simulink model "snap_adc5g_spec_rpi"  (R2019a)
settings: Solver=VariableStepDiscrete  StartTime=0.0  StopTime=10.0  RelTol=1e-3
undefined symbols (not defined in the file): pfb_coeff_gen_calc
libraries: xbsIndex_r4 x13965, casper_library_misc x80, casper_library_delays x43, xps_library x5, xbsReplacements_r4 x2, casper_library_communications x1
(part 2 of 152)

== system snap_adc5g_spec_rpi/fft_shift ==
  sim_1 : Inport
  convert1_1 : DataTypeConversion  OutDataTypeStr=fixdt('ufix32_En0')  LockScale=on
  convert2_1 : DataTypeConversion  OutDataTypeStr=fixdt('ufix32_En0')  ConvertRealWorld=Stored Integer (SI)  LockScale=on
  gain_1 : Gain
  io_delay : xbsIndex_r4/Delay  rst=off  infoeditControl=Selection of Reset will increase slice count due to use of real FFs and instead of SRLs  en=off  latency=0  reg_retiming=on  dbl_ovrd=off  block_type=delay
  reint1 : xbsIndex_r4/Reinterpret  force_arith_type=on  arith_type=Unsigned  force_bin_pt=on  bin_pt=0  block_type=reinterpret
  slice_reg : xbsIndex_r4/Slice  nbits=32  boolean_output=off  mode=Lower Bit Location + Width  bit1=0  base1=MSB of Input  bit0=0  base0=LSB of Input  dbl_ovrd=off  block_type=slice
  snap_adc5g_spec_rpi_fft_shift_user_data_out : xbsIndex_r4/Gateway In  gui_display_data_type=Fixed-point  arith_type=Unsigned  n_bits=32  bin_pt=0  preci_type=Single  exp_width=8  frac_width=24  rows=1  columns=1  quantization="Round  (unbiased: +/- Inf)"  overflow=Saturate  period=1  UseAsADC=off  ADCChannel='1'  interface=None  automatic_assignment=on  address_offset=hex2dec('00')  intf_name=''  intf_description=''  default_value=0  timing_constraint=None  locs_specified=off  LOCs={}  io_standard={}  inherit_from_input=off  hdl_port=on  dbl_ovrd=off  block_type=gatewayin
  in_reg : Outport
  wires:
  snap_adc5g_spec_rpi_fft_shift_user_data_out/1 -> io_delay/1
  sim_1/1 -> convert1_1/1
  convert1_1/1 -> convert2_1/1
  convert2_1/1 -> gain_1/1
  gain_1/1 -> snap_adc5g_spec_rpi_fft_shift_user_data_out/1
  io_delay/1 -> slice_reg/1
  slice_reg/1 -> reint1/1
  reint1/1 -> in_reg/1

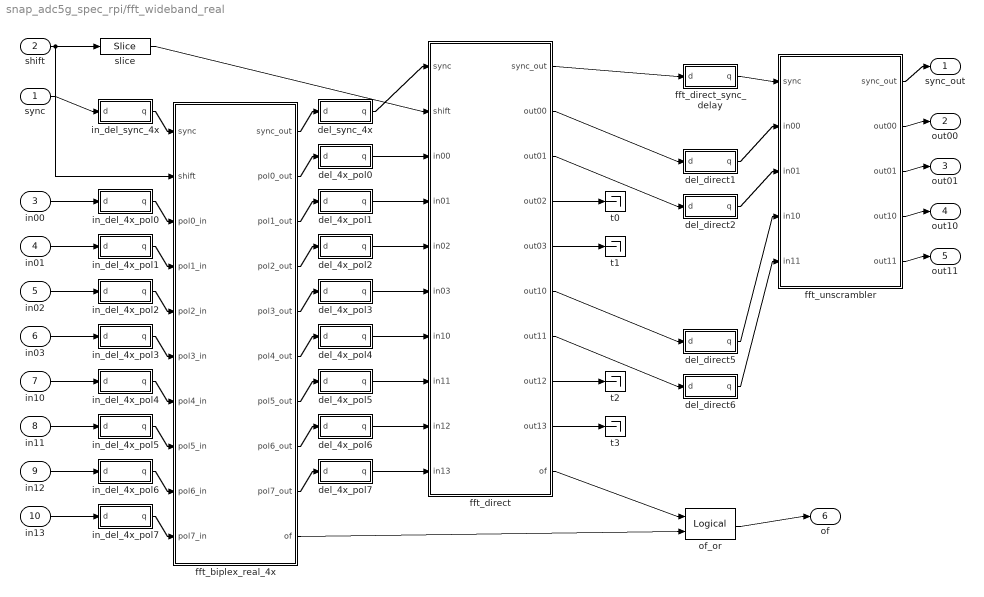
== system snap_adc5g_spec_rpi/fft_wideband_real ==
  sync : Inport
  shift : Inport  Port=2
  in00 : Inport  Port=3
  in01 : Inport  Port=4
  in02 : Inport  Port=5
  in03 : Inport  Port=6
  in10 : Inport  Port=7
  in11 : Inport  Port=8
  in12 : Inport  Port=9
  in13 : Inport  Port=10
  del_4x_pol0 : Subsystem  AncestorBlock=casper_library_delays/pipeline  mask(pipeline){csp_latency=0}
      mask prompts: csp_latency "Latency"
      mask help:
      | An explicitly laid-out delay line to avoid mapping to SRL16s
      | for use in pipelining to help achieve timing closure.
      mask init:
      | pipeline_init(gcb,'latency',csp_latency);
      settings: AttributesFormatString=Latency = %<latency>
      mask Display:
      | port_label('input', 1, 'd');
      | port_label('output', 1, 'q');
      | disp(['Z^-', num2str(csp_latency)]);
  del_4x_pol1 : Subsystem  AncestorBlock=casper_library_delays/pipeline  mask(pipeline){csp_latency=0}
      mask prompts: csp_latency "Latency"
      mask help:
      | An explicitly laid-out delay line to avoid mapping to SRL16s
      | for use in pipelining to help achieve timing closure.
      mask init:
      | pipeline_init(gcb,'latency',csp_latency);
      settings: AttributesFormatString=Latency = %<latency>
      mask Display:
      | port_label('input', 1, 'd');
      | port_label('output', 1, 'q');
      | disp(['Z^-', num2str(csp_latency)]);
  del_4x_pol2 : Subsystem  AncestorBlock=casper_library_delays/pipeline  mask(pipeline){csp_latency=0}
      mask prompts: csp_latency "Latency"
      mask help:
      | An explicitly laid-out delay line to avoid mapping to SRL16s
      | for use in pipelining to help achieve timing closure.
      mask init:
      | pipeline_init(gcb,'latency',csp_latency);
      settings: AttributesFormatString=Latency = %<latency>
      mask Display:
      | port_label('input', 1, 'd');
      | port_label('output', 1, 'q');
      | disp(['Z^-', num2str(csp_latency)]);
  del_4x_pol3 : Subsystem  AncestorBlock=casper_library_delays/pipeline  mask(pipeline){csp_latency=0}
      mask prompts: csp_latency "Latency"
      mask help:
      | An explicitly laid-out delay line to avoid mapping to SRL16s
      | for use in pipelining to help achieve timing closure.
      mask init:
      | pipeline_init(gcb,'latency',csp_latency);
      settings: AttributesFormatString=Latency = %<latency>
      mask Display:
      | port_label('input', 1, 'd');
      | port_label('output', 1, 'q');
      | disp(['Z^-', num2str(csp_latency)]);
  del_4x_pol4 : Subsystem  AncestorBlock=casper_library_delays/pipeline  mask(pipeline){csp_latency=0}
      mask prompts: csp_latency "Latency"
      mask help:
      | An explicitly laid-out delay line to avoid mapping to SRL16s
      | for use in pipelining to help achieve timing closure.
      mask init:
      | pipeline_init(gcb,'latency',csp_latency);
      settings: AttributesFormatString=Latency = %<latency>
      mask Display:
      | port_label('input', 1, 'd');
      | port_label('output', 1, 'q');
      | disp(['Z^-', num2str(csp_latency)]);
  del_4x_pol5 : Subsystem  AncestorBlock=casper_library_delays/pipeline  mask(pipeline){csp_latency=0}
      mask prompts: csp_latency "Latency"
      mask help:
      | An explicitly laid-out delay line to avoid mapping to SRL16s
      | for use in pipelining to help achieve timing closure.
      mask init:
      | pipeline_init(gcb,'latency',csp_latency);
      settings: AttributesFormatString=Latency = %<latency>
      mask Display:
      | port_label('input', 1, 'd');
      | port_label('output', 1, 'q');
      | disp(['Z^-', num2str(csp_latency)]);
  del_4x_pol6 : Subsystem  AncestorBlock=casper_library_delays/pipeline  mask(pipeline){csp_latency=0}
      mask prompts: csp_latency "Latency"
      mask help:
      | An explicitly laid-out delay line to avoid mapping to SRL16s
      | for use in pipelining to help achieve timing closure.
      mask init:
      | pipeline_init(gcb,'latency',csp_latency);
      settings: AttributesFormatString=Latency = %<latency>
      mask Display:
      | port_label('input', 1, 'd');
      | port_label('output', 1, 'q');
      | disp(['Z^-', num2str(csp_latency)]);
  del_4x_pol7 : Subsystem  AncestorBlock=casper_library_delays/pipeline  mask(pipeline){csp_latency=0}
      mask prompts: csp_latency "Latency"
      mask help:
      | An explicitly laid-out delay line to avoid mapping to SRL16s
      | for use in pipelining to help achieve timing closure.
      mask init:
      | pipeline_init(gcb,'latency',csp_latency);
      settings: AttributesFormatString=Latency = %<latency>
      mask Display:
      | port_label('input', 1, 'd');
      | port_label('output', 1, 'q');
      | disp(['Z^-', num2str(csp_latency)]);
  del_direct1 : Subsystem  AncestorBlock=casper_library_delays/pipeline  mask(pipeline){csp_latency=0}
      mask prompts: csp_latency "Latency"
      mask help:
      | An explicitly laid-out delay line to avoid mapping to SRL16s
      | for use in pipelining to help achieve timing closure.
      mask init:
      | pipeline_init(gcb,'latency',csp_latency);
      settings: AttributesFormatString=Latency = %<latency>
      mask Display:
      | port_label('input', 1, 'd');
      | port_label('output', 1, 'q');
      | disp(['Z^-', num2str(csp_latency)]);
  del_direct2 : Subsystem  AncestorBlock=casper_library_delays/pipeline  mask(pipeline){csp_latency=0}
      mask prompts: csp_latency "Latency"
      mask help:
      | An explicitly laid-out delay line to avoid mapping to SRL16s
      | for use in pipelining to help achieve timing closure.
      mask init:
      | pipeline_init(gcb,'latency',csp_latency);
      settings: AttributesFormatString=Latency = %<latency>
      mask Display:
      | port_label('input', 1, 'd');
      | port_label('output', 1, 'q');
      | disp(['Z^-', num2str(csp_latency)]);
  del_direct5 : Subsystem  AncestorBlock=casper_library_delays/pipeline  mask(pipeline){csp_latency=0}
      mask prompts: csp_latency "Latency"
      mask help:
      | An explicitly laid-out delay line to avoid mapping to SRL16s
      | for use in pipelining to help achieve timing closure.
      mask init:
      | pipeline_init(gcb,'latency',csp_latency);
      settings: AttributesFormatString=Latency = %<latency>
      mask Display:
      | port_label('input', 1, 'd');
      | port_label('output', 1, 'q');
      | disp(['Z^-', num2str(csp_latency)]);
  del_direct6 : Subsystem  AncestorBlock=casper_library_delays/pipeline  mask(pipeline){csp_latency=0}
      mask prompts: csp_latency "Latency"
      mask help:
      | An explicitly laid-out delay line to avoid mapping to SRL16s
      | for use in pipelining to help achieve timing closure.
      mask init:
      | pipeline_init(gcb,'latency',csp_latency);
      settings: AttributesFormatString=Latency = %<latency>
      mask Display:
      | port_label('input', 1, 'd');
      | port_label('output', 1, 'q');
      | disp(['Z^-', num2str(csp_latency)]);
  del_sync_4x : Subsystem  AncestorBlock=casper_library_delays/pipeline  mask(pipeline){csp_latency=0}
      mask prompts: csp_latency "Latency"
      mask help:
      | An explicitly laid-out delay line to avoid mapping to SRL16s
      | for use in pipelining to help achieve timing closure.
      mask init:
      | pipeline_init(gcb,'latency',csp_latency);
      settings: AttributesFormatString=Latency = %<latency>
      mask Display:
      | port_label('input', 1, 'd');
      | port_label('output', 1, 'q');
      | disp(['Z^-', num2str(csp_latency)]);
  fft_biplex_real_4x : Subsystem  Tag=casper:fft_biplex_real_4x  AncestorBlock=casper_library_ffts/fft_biplex_real_4x  mask(fft_biplex_real_4x){n_inputs=2, FFTSize=11, input_bit_width=18, bin_pt_in=17, coeff_bit_width=18, async=off, floating_point=off, float_type=single, exp_width=8, frac_width=24, add_latency=1, mult_latency=2, bram_latency=3, conv_latency=1, add_pipe_latency=0, mult_pipe_latency=0, quantization=Round  (unbiased: Even Values), overflow=Wrap, delays_bit_limit=8, coeffs_bit_limit=9, coeff_sharing=on, coeff_decimation=on, max_fanout=4, mult_spec=[2 2 2 2 2 2 2 2 2 2 2], bitgrowth=off, max_bits=19, hardcode_shifts=off, shift_schedule=[1 1 1 1 1 1 1 1 1 1 1], dsp48_adders=off}
      mask prompts: n_inputs "Number simultaneous inputs (4*?)"; FFTSize "Size of FFT: (2^? pts)"; input_bit_width "Input bit width"; bin_pt_in "Input binary point"; coeff_bit_width "Coefficient Bit Width"; async "Asynchronous operation"; floating_point "floating point"; float_type "float type"; exp_width "exponent width"; frac_width "fraction width"; add_latency "Add Latency"; mult_latency "Mult Latency"; bram_latency "BRAM Latency"; conv_latency "Convert latency"; add_pipe_latency "Add Interface Pipeline Latency"; mult_pipe_latency "CMult Pipeline Latency"; quantization "Quantization Behavior"; overflow "Overflow Behavior"; delays_bit_limit "Number bits above which to implement stage's delays in BRAM (2^? bits)"; coeffs_bit_limit "Number bits above which to store stage's coefficients in BRAM (2^? bits)"; coeff_sharing "BRAM sharing in coeff storage"; coeff_decimation "Store a fraction of coeff factors where useful"; max_fanout "Maximum fanout"; mult_spec "Multiplier impl. (0=core, 1=embedded, 2=behavioural) (left=1st stage, or just one value)"; bitgrowth "Bitgrowth instead of shifting"; max_bits "Max bits to grow to"; hardcode_shifts "Hardcode shift schedule"; shift_schedule "Shift schedule"; dsp48_adders "DSP48 adders in butterfly"
      mask help: A real-sampled biplex FFT, with output demuxed by 4.
      mask init:
      | fft_biplex_real_4x_init(gcb, ...
      |     'n_inputs', n_inputs, ...
      |     'FFTSize', FFTSize, ...
      |     'input_bit_width', input_bit_width, ...
      |     'bin_pt_in', bin_pt_in, ...
      |     'coeff_bit_width', coeff_bit_width, ...
      |     'floating_point', floating_point, ...
      |     'float_type', float_type, ...
      |     'exp_width', exp_width, ...
      |     'frac_width', frac_width, ...    
      |     'async', async, ...
      |     'add_latency', add_latency, ...
      |     'mult_latency', mult_latency, ...
      |     'bram_latency', bram_latency, ...
      |     'conv_latency', conv_latency, ...
      |     'add_pipe_latency', add_pipe_latency, ...
      |     'mult_pipe_latency', mult_pipe_latency, ...    
      |     'quantization', quantization, ...
      |     'overflow', overflow, ...
      |     'delays_bit_limit', delays_bit_limit, ... 
      |     'coeffs_bit_limit', coeffs_bit_limit, ...
      |     'coeff_sharing', coeff_sharing, ...
      |     'coeff_decimation', coeff_decimation, ...
      |     'max_fanout', max_fanout, ...   
      |     'mult_spec', mult_spec, ...
      |     'bitgrowth', bitgrowth, ...
      |     'max_bits', max_bits, ...
      |     'hardcode_shifts', hardcode_shifts, ...
      |     'shift_schedule', shift_schedule, ...
      |     'dsp48_adders', dsp48_adders);
      settings: AttributesFormatString=|
      | 11 stages
      | [18,18]
      | Round  (unbiased: Even Values)
      | Wrap
      mask Help: eval('xlWeb(''http://casper.berkeley.edu/wiki/Fft_biplex_real_4x'')')
      mask Callback floating_point:
      | onoff = get_param(gcb, 'floating_point');
      | if strcmp(onoff,'on')
      |     enable_fixpt = 'off'
      |     set_param_state(gcb, 'float_type', 'on')
      | 
      |     f_type = get_param(gcb, 'float_type')
      |     if strcmp(f_type,'custom')
      |        set_param_state(gcb, 'exp_width', 'on')
      |        set_param_state(gcb, 'frac_width', 'on')
      |     else
      |        set_param_state(gcb, 'exp_width', 'off')
      |        set_param_state(gcb, 'frac_width', 'off')
      |     end
      | 
      | 
      | else
      |     enable_fixpt = 'on'
      |     set_param_state(gcb, 'float_type', 'off')
      |     set_param_state(gcb, 'exp_width', 'off')
      |     set_param_state(gcb, 'frac_width', 'off')
      | end
      | 
      | set_param_state(gcb, 'input_bit_width', enable_fixpt)
      | set_param_state(gcb, 'bin_pt_in', enable_fixpt)
      | set_param_state(gcb, 'coeff_bit_width', enable_fixpt)
      mask TypeOptions float_type: single | custom
      mask Callback float_type:
      | f_type = get_param(gcb, 'float_type')
      | if strcmp(f_type,'custom')
      |     set_param_state(gcb, 'exp_width', 'on')
      |     set_param_state(gcb, 'frac_width', 'on')
      | else
      |     set_param_state(gcb, 'exp_width', 'off')
      |     set_param_state(gcb, 'frac_width', 'off')
      | end
      mask TypeOptions quantization: Truncate | Round  (unbiased: +/- Inf) | Round  (unbiased: Even Values)
      mask TypeOptions overflow: Wrap | Saturate | Error
      mask Callback hardcode_shifts:
      | hardcode_shifts = get_param(gcb, 'hardcode_shifts');
      | set_param_state(gcb, 'shift_schedule', hardcode_shifts);
      mask Callback dsp48_adders: fft_callback_dsp48_adders(gcb);
      mask DialogControl ParameterTabVar0 Prompt: Basic
      mask DialogControl ParameterTabVar01 Prompt: Latency
      mask DialogControl ParameterTabVar012 Prompt: Implementation
  fft_direct : Subsystem  AncestorBlock=casper_library_ffts/fft_direct  mask(fft_direct){n_streams=2, FFTSize=2, input_bit_width=18, bin_pt_in=17, coeff_bit_width=18, map_tail=on, LargerFFTSize=13, StartStage=12, async=off, floating_point=off, float_type=single, exp_width=8, frac_width=24, add_latency=1, mult_latency=2, bram_latency=3, conv_latency=1, add_pipe_latency=0, mult_pipe_latency=0, quantization=Round  (unbiased: Even Values), overflow=Wrap, coeffs_bit_limit=9, coeff_sharing=on, coeff_decimation=on, coeff_generation=off, cal_bits=1, n_bits_rotation=25, max_fanout=4, mult_spec=[2 2], bitgrowth=off, max_bits=19, hardcode_shifts=off, shift_schedule=[1 1], dsp48_adders=off}
      mask prompts: n_streams "Number simultaneous streams"; FFTSize "Size of FFT: (2^? pts)"; input_bit_width "Input Bit Width"; bin_pt_in "Input binary point"; coeff_bit_width "Coefficient Bit Width"; map_tail "Map Tail of Larger FFT"; LargerFFTSize "Size of Larger FFT (2^?)"; StartStage "Start Stage of Map Tail"; async "Asynchronous operation"; floating_point "floating point"; exp_width "exponent width"; frac_width "fraction width"; add_latency "Add Latency"; mult_latency "Mult Latency"; bram_latency "BRAM Latency"; conv_latency "Convert latency"; add_pipe_latency "Add interface pipeline latency"; mult_pipe_latency "Cmult pipeline latency"; quantization "Quantization Behavior"; overflow "Overflow Behavior"; coeffs_bit_limit "Number bits above which to store stage's coefficients in BRAM (2^? bits)"; coeff_sharing "BRAM sharing in coeff storage"; coeff_decimation "Store a fraction of coeff factors where useful"; coeff_generation "Generate coeffs with multipliers where useful"; cal_bits "Number calibration locations when generating coeffs (2^?)"; n_bits_rotation "Feedback rotation vector resolution"; max_fanout "Maximum fanout"; mult_spec "Multiplier impl. (0=core, 1=embedded, 2=behavioural) (left=1st stage, or just one value)"; bitgrowth "Bit growth instead of shifting"; max_bits "Max bits to growth to"; hardcode_shifts "Hardcode shift schedule"; shift_schedule "Shift schedule"; dsp48_adders "DSP48 adders in butterfly"
      mask help:
      | FFT internal block.
      |
      | Implements an N-point FFT as the classic butterfly structure,
      | with N inputs and N outputs.
      mask init:
      | fft_direct_init(gcb, ...
      |     'n_streams', n_streams, ...
      |     'FFTSize', FFTSize, ...
      |     'input_bit_width', input_bit_width, ...
      |     'bin_pt_in', bin_pt_in, ...
      |     'coeff_bit_width', coeff_bit_width, ...
      |     'map_tail', map_tail, ...
      |     'LargerFFTSize', LargerFFTSize, ...
      |     'StartStage', StartStage, ...
      |     'async', async, ...
      |     'add_latency', add_latency, ...
      |     'mult_latency', mult_latency, ...
      |     'bram_latency', bram_latency, ...
      |     'conv_latency', conv_latency, ...
      |     'add_pipe_latency', add_pipe_latency, ...
      |     'mult_pipe_latency', mult_pipe_latency, ...          
      |     'quantization', quantization, ...
      |     'overflow', overflow, ...
      |     'coeffs_bit_limit', coeffs_bit_limit, ...
      |     'coeff_sharing', coeff_sharing, ...
      |     'coeff_decimation', coeff_decimation, ...
      |     'coeff_generation', coeff_generation, ...
      |     'floating_point', floating_point, ...
      |     'float_type', float_type, ...
      |     'exp_width', exp_width, ...
      |     'frac_width', frac_width, ...      
      |     'cal_bits', cal_bits, ...
      |     'n_bits_rotation', n_bits_rotation, ...
      |     'max_fanout', max_fanout, ...
      |     'mult_spec', mult_spec, ...
      |     'bitgrowth', bitgrowth, ...
      |     'max_bits', max_bits, ...
      |     'hardcode_shifts', hardcode_shifts, ...
      |     'shift_schedule', shift_schedule, ...
      |     'dsp48_adders', dsp48_adders);
      settings: AttributesFormatString=|
      | stages [12:13] of 13
      | [18,18]
      | Round  (unbiased: Even Values)
      | Wrap
      mask Callback map_tail:
      | map_tail = get_param(gcb, 'map_tail');
      | set_param_state(gcb, 'LargerFFTSize', map_tail);
      | set_param_state(gcb, 'StartStage', map_tail);
      mask Callback floating_point:
      | onoff = get_param(gcb, 'floating_point');
      | if strcmp(onoff,'on')
      |     enable_fixpt = 'off'
      |     set_param_state(gcb, 'float_type', 'on')
      | 
      |     f_type = get_param(gcb, 'float_type')
      |     if strcmp(f_type,'custom')
      |         set_param_state(gcb, 'exp_width', 'on')
      |         set_param_state(gcb, 'frac_width', 'on')
      |     else
      |         set_param_state(gcb, 'exp_width', 'off')
      |         set_param_state(gcb, 'frac_width', 'off')
      |     end
      | 
      | 
      | else
      |     enable_fixpt = 'on'
      |     set_param_state(gcb, 'float_type', 'off')
      |     set_param_state(gcb, 'exp_width', 'off')
      |     set_param_state(gcb, 'frac_width', 'off')
      | end
      | 
      | set_param_state(gcb, 'input_bit_width', enable_fixpt)
      | set_param_state(gcb, 'bin_pt_in', enable_fixpt)
      | set_param_state(gcb, 'coeff_bit_width', enable_fixpt)
      mask TypeOptions float_type: single | custom
      mask Callback float_type:
      | f_type = get_param(gcb, 'float_type')
      | if strcmp(f_type,'custom')
      |     set_param_state(gcb, 'exp_width', 'on')
      |     set_param_state(gcb, 'frac_width', 'on')
      | else
      |     set_param_state(gcb, 'exp_width', 'off')
      |     set_param_state(gcb, 'frac_width', 'off')
      | end
      mask TypeOptions quantization: Truncate | Round  (unbiased: +/- Inf) | Round  (unbiased: Even Values)
      mask TypeOptions overflow: Wrap | Saturate | Error
      mask Callback hardcode_shifts:
      | hardcode_shifts = get_param(gcb, 'hardcode_shifts');
      | set_param_state(gcb, 'shift_schedule', hardcode_shifts);
      mask Callback dsp48_adders: fft_callback_dsp48_adders(gcb);
      mask DialogControl ParameterTabVar0 Prompt: Basic
      mask DialogControl ParameterTabVar01 Prompt: Latency
      mask DialogControl ParameterTabVar012 Prompt: Implementation
  fft_direct_sync_delay : Subsystem  AncestorBlock=casper_library_delays/pipeline  mask(pipeline){csp_latency=0}
      mask prompts: csp_latency "Latency"
      mask help:
      | An explicitly laid-out delay line to avoid mapping to SRL16s
      | for use in pipelining to help achieve timing closure.
      mask init:
      | pipeline_init(gcb,'latency',csp_latency);
      settings: AttributesFormatString=Latency = %<latency>
      mask Display:
      | port_label('input', 1, 'd');
      | port_label('output', 1, 'q');
      | disp(['Z^-', num2str(csp_latency)]);
  fft_unscrambler : Subsystem  AncestorBlock=casper_library_ffts/fft_unscrambler  mask(fft_unscrambler){n_streams=2, FFTSize=12, n_inputs=1, n_bits_in=18, bram_latency=3, coeffs_bit_limit=9, async=off, floating_point=off, float_type=single, exp_width=8, frac_width=24}
      mask prompts: n_streams "Number of simultaneous streams"; FFTSize "Size of FFT: (2^?)"; n_inputs "Number of simultaneous inputs: (2^?)"; n_bits_in "Input bit width"; bram_latency "BRAM Latency"; coeffs_bit_limit "Number bits above which to store map coefficients in BRAM (2^? bits)"; async "Asynchronous operation"; floating_point "floating point"; float_type "float type"; exp_width "exponent width"; frac_width "fraction width"
      mask init:
      | fft_unscrambler_init(gcb, ...
      |     'n_streams', n_streams, ...
      |     'FFTSize',FFTSize, ... 
      |     'n_inputs', n_inputs, ...
      |     'n_bits_in', n_bits_in, ...
      |     'floating_point', floating_point, ...
      |     'float_type', float_type, ...
      |     'exp_width', exp_width, ...
      |     'frac_width', frac_width, ...    
      |     'bram_latency', bram_latency, ...
      |     'coeffs_bit_limit', coeffs_bit_limit, ...
      |     'async', async);
      settings: AttributesFormatString=FFTSize=12, n_inputs=1
      mask Callback floating_point:
      | onoff = get_param(gcb, 'floating_point');
      | if strcmp(onoff,'on')
      |     enable_fixpt = 'off'
      |     set_param_state(gcb, 'float_type', 'on')
      | 
      |     f_type = get_param(gcb, 'float_type')
      |     if strcmp(f_type,'custom')
      |         set_param_state(gcb, 'exp_width', 'on')
      |         set_param_state(gcb, 'frac_width', 'on')
      |     else
      |         set_param_state(gcb, 'exp_width', 'off')
      |         set_param_state(gcb, 'frac_width', 'off')
      |     end
      | 
      | 
      | else
      |     enable_fixpt = 'on'
      |     set_param_state(gcb, 'float_type', 'off')
      |     set_param_state(gcb, 'exp_width', 'off')
      |     set_param_state(gcb, 'frac_width', 'off')
      | end
      | 
      | set_param_state(gcb, 'n_bits_in', enable_fixpt)
      mask TypeOptions float_type: single | custom
      mask Callback float_type:
      | f_type = get_param(gcb, 'float_type')
      | if strcmp(f_type,'custom')
      |     set_param_state(gcb, 'exp_width', 'on')
      |     set_param_state(gcb, 'frac_width', 'on')
      | else
      |     set_param_state(gcb, 'exp_width', 'off')
      |     set_param_state(gcb, 'frac_width', 'off')
      | end
  in_del_4x_pol0 : Subsystem  AncestorBlock=casper_library_delays/pipeline  mask(pipeline){csp_latency=0}
      mask prompts: csp_latency "Latency"
      mask help:
      | An explicitly laid-out delay line to avoid mapping to SRL16s
      | for use in pipelining to help achieve timing closure.
      mask init:
      | pipeline_init(gcb,'latency',csp_latency);
      settings: AttributesFormatString=Latency = %<latency>
      mask Display:
      | port_label('input', 1, 'd');
      | port_label('output', 1, 'q');
      | disp(['Z^-', num2str(csp_latency)]);
  in_del_4x_pol1 : Subsystem  AncestorBlock=casper_library_delays/pipeline  mask(pipeline){csp_latency=0}
      mask prompts: csp_latency "Latency"
      mask help:
      | An explicitly laid-out delay line to avoid mapping to SRL16s
      | for use in pipelining to help achieve timing closure.
      mask init:
      | pipeline_init(gcb,'latency',csp_latency);
      settings: AttributesFormatString=Latency = %<latency>
      mask Display:
      | port_label('input', 1, 'd');
      | port_label('output', 1, 'q');
      | disp(['Z^-', num2str(csp_latency)]);
  in_del_4x_pol2 : Subsystem  AncestorBlock=casper_library_delays/pipeline  mask(pipeline){csp_latency=0}
      mask prompts: csp_latency "Latency"
      mask help:
      | An explicitly laid-out delay line to avoid mapping to SRL16s
      | for use in pipelining to help achieve timing closure.
      mask init:
      | pipeline_init(gcb,'latency',csp_latency);
      settings: AttributesFormatString=Latency = %<latency>
      mask Display:
      | port_label('input', 1, 'd');
      | port_label('output', 1, 'q');
      | disp(['Z^-', num2str(csp_latency)]);
  in_del_4x_pol3 : Subsystem  AncestorBlock=casper_library_delays/pipeline  mask(pipeline){csp_latency=0}
      mask prompts: csp_latency "Latency"
      mask help:
      | An explicitly laid-out delay line to avoid mapping to SRL16s
      | for use in pipelining to help achieve timing closure.
      mask init:
      | pipeline_init(gcb,'latency',csp_latency);
      settings: AttributesFormatString=Latency = %<latency>
      mask Display:
      | port_label('input', 1, 'd');
      | port_label('output', 1, 'q');
      | disp(['Z^-', num2str(csp_latency)]);
  in_del_4x_pol4 : Subsystem  AncestorBlock=casper_library_delays/pipeline  mask(pipeline){csp_latency=0}
      mask prompts: csp_latency "Latency"
      mask help:
      | An explicitly laid-out delay line to avoid mapping to SRL16s
      | for use in pipelining to help achieve timing closure.
      mask init:
      | pipeline_init(gcb,'latency',csp_latency);
      settings: AttributesFormatString=Latency = %<latency>
      mask Display:
      | port_label('input', 1, 'd');
      | port_label('output', 1, 'q');
      | disp(['Z^-', num2str(csp_latency)]);
  in_del_4x_pol5 : Subsystem  AncestorBlock=casper_library_delays/pipeline  mask(pipeline){csp_latency=0}
      mask prompts: csp_latency "Latency"
      mask help:
      | An explicitly laid-out delay line to avoid mapping to SRL16s
      | for use in pipelining to help achieve timing closure.
      mask init:
      | pipeline_init(gcb,'latency',csp_latency);
      settings: AttributesFormatString=Latency = %<latency>
      mask Display:
      | port_label('input', 1, 'd');
      | port_label('output', 1, 'q');
      | disp(['Z^-', num2str(csp_latency)]);
  in_del_4x_pol6 : Subsystem  AncestorBlock=casper_library_delays/pipeline  mask(pipeline){csp_latency=0}
      mask prompts: csp_latency "Latency"
      mask help:
      | An explicitly laid-out delay line to avoid mapping to SRL16s
      | for use in pipelining to help achieve timing closure.
      mask init:
      | pipeline_init(gcb,'latency',csp_latency);
      settings: AttributesFormatString=Latency = %<latency>
      mask Display:
      | port_label('input', 1, 'd');
      | port_label('output', 1, 'q');
      | disp(['Z^-', num2str(csp_latency)]);
  in_del_4x_pol7 : Subsystem  AncestorBlock=casper_library_delays/pipeline  mask(pipeline){csp_latency=0}
      mask prompts: csp_latency "Latency"
      mask help:
      | An explicitly laid-out delay line to avoid mapping to SRL16s
      | for use in pipelining to help achieve timing closure.
      mask init:
      | pipeline_init(gcb,'latency',csp_latency);
      settings: AttributesFormatString=Latency = %<latency>
      mask Display:
      | port_label('input', 1, 'd');
      | port_label('output', 1, 'q');
      | disp(['Z^-', num2str(csp_latency)]);
  in_del_sync_4x : Subsystem  AncestorBlock=casper_library_delays/pipeline  mask(pipeline){csp_latency=0}
      mask prompts: csp_latency "Latency"
      mask help:
      | An explicitly laid-out delay line to avoid mapping to SRL16s
      | for use in pipelining to help achieve timing closure.
      mask init:
      | pipeline_init(gcb,'latency',csp_latency);
      settings: AttributesFormatString=Latency = %<latency>
      mask Display:
      | port_label('input', 1, 'd');
      | port_label('output', 1, 'q');
      | disp(['Z^-', num2str(csp_latency)]);
  of_or : xbsIndex_r4/Logical  logical_function=OR  inputs=2  en=off  latency=1  precision=Full  arith_type=Unsigned  n_bits=16  bin_pt=0  align_bp=on  dbl_ovrd=off  block_type=logical
  slice : xbsIndex_r4/Slice  nbits=2  boolean_output=off  mode=Lower Bit Location + Width  bit1=0  base1=MSB of Input  bit0=11  base0=LSB of Input  dbl_ovrd=off  block_type=slice
  t{0..3} (4 alike) : Terminator
  sync_out : Outport
  out00 : Outport  Port=2
  out01 : Outport  Port=3
  out10 : Outport  Port=4
  out11 : Outport  Port=5
  of : Outport  Port=6
  wires:
  sync/1 -> in_del_sync_4x/1(d)
  shift/1 -> fft_biplex_real_4x/2(shift), slice/1
  in_del_sync_4x/1(q) -> fft_biplex_real_4x/1(sync)
  fft_biplex_real_4x/1(sync_out) -> del_sync_4x/1(d)
  del_sync_4x/1(q) -> fft_direct/1(sync)
  fft_direct/4(out02) -> t0/1
  fft_direct/5(out03) -> t1/1
  fft_direct/8(out12) -> t2/1
  fft_direct/9(out13) -> t3/1
  fft_direct/1(sync_out) -> fft_direct_sync_delay/1(d)
  fft_direct_sync_delay/1(q) -> fft_unscrambler/1(sync)
  fft_unscrambler/1(sync_out) -> sync_out/1
  fft_direct/2(out00) -> del_direct1/1(d)
  del_direct1/1(q) -> fft_unscrambler/2(in00)
  fft_unscrambler/2(out00) -> out00/1
  fft_direct/3(out01) -> del_direct2/1(d)
  del_direct2/1(q) -> fft_unscrambler/3(in01)
  fft_unscrambler/3(out01) -> out01/1
  fft_direct/6(out10) -> del_direct5/1(d)
  del_direct5/1(q) -> fft_unscrambler/4(in10)
  fft_unscrambler/4(out10) -> out10/1
  fft_direct/7(out11) -> del_direct6/1(d)
  del_direct6/1(q) -> fft_unscrambler/5(in11)
  fft_unscrambler/5(out11) -> out11/1
  slice/1 -> fft_direct/2(shift)
  fft_biplex_real_4x/10(of) -> of_or/2
  fft_direct/10(of) -> of_or/1
  of_or/1 -> of/1
  in00/1 -> in_del_4x_pol0/1(d)
  in_del_4x_pol0/1(q) -> fft_biplex_real_4x/3(pol0_in)
  fft_biplex_real_4x/2(pol0_out) -> del_4x_pol0/1(d)
  del_4x_pol0/1(q) -> fft_direct/3(in00)
  in01/1 -> in_del_4x_pol1/1(d)
  in_del_4x_pol1/1(q) -> fft_biplex_real_4x/4(pol1_in)
  fft_biplex_real_4x/3(pol1_out) -> del_4x_pol1/1(d)
  del_4x_pol1/1(q) -> fft_direct/4(in01)
  in02/1 -> in_del_4x_pol2/1(d)
  in_del_4x_pol2/1(q) -> fft_biplex_real_4x/5(pol2_in)
  fft_biplex_real_4x/4(pol2_out) -> del_4x_pol2/1(d)
  del_4x_pol2/1(q) -> fft_direct/5(in02)
  in03/1 -> in_del_4x_pol3/1(d)
  in_del_4x_pol3/1(q) -> fft_biplex_real_4x/6(pol3_in)
  fft_biplex_real_4x/5(pol3_out) -> del_4x_pol3/1(d)
  del_4x_pol3/1(q) -> fft_direct/6(in03)
  in10/1 -> in_del_4x_pol4/1(d)
  in_del_4x_pol4/1(q) -> fft_biplex_real_4x/7(pol4_in)
  fft_biplex_real_4x/6(pol4_out) -> del_4x_pol4/1(d)
  del_4x_pol4/1(q) -> fft_direct/7(in10)
  in11/1 -> in_del_4x_pol5/1(d)
  in_del_4x_pol5/1(q) -> fft_biplex_real_4x/8(pol5_in)
  fft_biplex_real_4x/7(pol5_out) -> del_4x_pol5/1(d)
  del_4x_pol5/1(q) -> fft_direct/8(in11)
  in12/1 -> in_del_4x_pol6/1(d)
  in_del_4x_pol6/1(q) -> fft_biplex_real_4x/9(pol6_in)
  fft_biplex_real_4x/8(pol6_out) -> del_4x_pol6/1(d)
  del_4x_pol6/1(q) -> fft_direct/9(in12)
  in13/1 -> in_del_4x_pol7/1(d)
  in_del_4x_pol7/1(q) -> fft_biplex_real_4x/10(pol7_in)
  fft_biplex_real_4x/9(pol7_out) -> del_4x_pol7/1(d)
  del_4x_pol7/1(q) -> fft_direct/10(in13)

== system snap_adc5g_spec_rpi/of_detect ==
  rst : Inport
  of : Inport  Port=2
  Constant : xbsIndex_r4/Constant  const=0  gui_display_data_type=Fixed-point  arith_type=Unsigned  n_bits=16  bin_pt=0  preci_type=Single  exp_width=8  frac_width=24  explicit_period=on  period=1  equ=P=C  opselect=C  inp2=PCIN>>17  opr=+  inp1=P  carry=CIN  dbl_ovrd=off  block_type=constant
  Register : xbsIndex_r4/Register  init=0  rst=on  en=on  dbl_ovrd=off  block_type=register
  Relational : xbsIndex_r4/Relational  mode=a!=b  op_type=Bool  en=off  latency=1  dbl_ovrd=off  block_type=relational
  err : Outport
  wires:
  Relational/1 -> Register/3, Register/1
  rst/1 -> Register/2
  Register/1 -> err/1
  Constant/1 -> Relational/2
  of/1 -> Relational/1
